simulink model "TV_FLC_V3_Codegen"  (R2026a)
settings: Solver=FixedStepDiscrete  StopTime=100  FixedStep=0.003  MaxStep=0.4  AbsTol=1e-3
model workspace (MAT data in the model file):
  Af = 1.20000004768
  C_alpha_F = 46504
  D = 11
  F = 0.0421790704131
  FIS_DYC_3 : fistree (value not decoded)
  Gain = 0.175131350756
  Gr = 5
  I = 6000
  Kp_TV_Beta : Simulink.Parameter (value not decoded)
  Kp_TV_Yaw : Simulink.Parameter (value not decoded)
  Ku = -0.000124337399029
  L = 1.57799994946
  Load_Ref = [0 400 500 600 700 800 900 1000 1100 1200 1300 1400 ... (18 elements, 18x1)]
  MotorT = [51.0306892395 51.0306892395 51.0306892395 51.0306892395 51.0306892395 51.0306892395 51.0306892395 51.0306892395 51.0306892395 51.0306892395 51.0306892395 51.0306892395 ... (47 elements, 1x47)]
  MotorW = [0 100 200 300 400 500 600 700 800 900 1000 1100 ... (47 elements, 1x47)]
  P = 800
  Slip_Ctrl_Kd : Simulink.Parameter (value not decoded)
  Slip_Ctrl_Ki : Simulink.Parameter (value not decoded)
  Slip_Ctrl_Kn : Simulink.Parameter (value not decoded)
  Slip_Ctrl_Kp : Simulink.Parameter (value not decoded)
  Slip_Ref = [0.151999995112 0.151999995112 0.151999995112 0.115999996662 0.101999998093 0.0960000008345 0.0920000001788 0.0900000035763 0.0900000035763 0.0900000035763 0.0939999967813 0.097999997437 ... (18 elements, 18x1)]
  Slip_Steer_th : Simulink.Parameter (value not decoded)
  Slip_TC_Enable : Simulink.Parameter (value not decoded)
  Tmax = 51.0306892395
  a = 0.823199987411
  a_cop = 0.707000017166
  cd = -2.15000009537
  g = 9.81000041962
  h_CG = 0.358300000429
  m = 320
  ro = 1.22599995136
  rwheel = 0.263000011444
  tr = 1.24800002575
  vx_th = 1
symbols that are objects in the model workspace (value not decoded): Kp_TV_Beta, Kp_TV_Yaw, Slip_Ctrl_Kd, Slip_Ctrl_Ki, Slip_Ctrl_Kn, Slip_Ctrl_Kp, Slip_Steer_th, Slip_TC_Enable
undefined symbols (not defined in the file or in its folder): dspblkCoreblockFVToolHelper, gcbh
libraries: simulink x5, sl_discontinuities x3, slpidlib x2, fuzblock x1
(part 2 of 2)

== system TV_FLC_V3_Codegen/Slip Control/Maximum Torque Allowed/Slip Correction Right ==
  Fz_rl : Inport  OutDataTypeStr=single
  kappa_rr : Inport  Port=2
  1-D Lookup Table : Lookup_n-D  NumberOfTableDimensions=1  BreakpointsForDimension1=Load_Ref  Table=Slip_Ref  ExtrapMethod=Clip  UseLastTableValue=on  InternalRulePriority=Speed  RndMeth=Simplest
  PID Controller : slpidlib/PID Controller  Controller=PID  Form=Parallel  TimeDomain=Discrete-time  UseExternalTs=off  SampleTime=0.003  IntegratorMethod=Forward Euler  FilterMethod=Forward Euler  ControllerParametersSource=internal  P=Slip_Ctrl_Kp  I=Slip_Ctrl_Ki  UseKiTs=off  D=Slip_Ctrl_Kd  UseExternalDerivativeSource=off  N=Slip_Ctrl_Kn  UseFilter=on  TunerSelectOption=Transfer Function Based (PID Tuner App)  InitialConditionSource=internal  InitialConditionForIntegrator=Tmax  InitialConditionForFilter=0  DifferentiatorICPrevScaledInput=Tmax  ExternalReset=none  TrackingMode=off  Kt=1  LimitOutput=on  SatLimitsSource=internal  UpperSaturationLimit=Tmax  LowerSaturationLimit=0  LinearizeAsGain=on  AntiWindupMode=clamping  Kb=1  LimitIntegrator=off  UpperIntegratorSaturationLimit=inf  LowerIntegratorSaturationLimit=-inf  POutMin=[]  POutMax=[]  IOutMin=[]  IOutMax=[]  DOutMin=[]  DOutMax=[]  NOutMin=[]  NOutMax=[]  SumOutMin=[]  SumOutMax=[]  SaturationOutMin=[]  SaturationOutMax=[]  PParamMin=[]  PParamMax=[]  IParamMin=[]  IParamMax=[]  DParamMin=[]  DParamMax=[]  NParamMin=[]  NParamMax=[]  KbParamMin=[]  KbParamMax=[]  KtParamMin=[]  KtParamMax=[]  KbOutMin=[]  KbOutMax=[]  KtOutMin=[]  KtOutMax=[]  IntegratorOutMin=[]  IntegratorOutMax=[]  FilterOutMin=[]  FilterOutMax=[]  SumI1OutMin=[]  SumI1OutMax=[]  SumI2OutMin=[]  SumI2OutMax=[]  SumI3OutMin=[]  SumI3OutMax=[]  SumI4OutMin=[]  SumI4OutMax=[]  SumDOutMin=[]  SumDOutMax=[]  DifferentiatorOutMin=[]  DifferentiatorOutMax=[]  FilterDiffOutCoefMin=[]  FilterDiffOutCoefMax=[]  ReciprocalOutMin=[]  ReciprocalOutMax=[]  SumDenOutMin=[]  SumDenOutMax=[]  SumNumOutMin=[]  SumNumOutMax=[]  DivideOutMin=[]  DivideOutMax=[]  UdiffTsProdOutMin=[]  UdiffTsProdOutMax=[]  NTsProdOutMin=[]  NTsProdOutMax=[]  UintegralTsProdOutMin=[]  UintegralTsProdOutMax=[]  UngainTsProdOutMin=[]  UngainTsProdOutMax=[]  ClampingZeroOutDataTypeStr=Inherit: Inherit via back propagation  ClampingZeroOutMin=[]  ClampingZeroOutMax=[]  FilterDenConstantOutDataTypeStr=Inherit: Inherit via back propagation  FilterDenConstantOutMin=[]  FilterDenConstantOutMax=[]  PCopyOutDataTypeStr=Inherit: Inherit via back propagation  PCopyOutMin=[]  PCopyOutMax=[]  NCopyOutDataTypeStr=Inherit: Inherit via back propagation  NCopyOutMin=[]  NCopyOutMax=[]  IntegratorContinuousStateAttributes=''  IntegratorStateMustResolveToSignalObject=off  IntegratorRTWStateStorageClass=Auto  FilterContinuousStateAttributes=''  FilterStateMustResolveToSignalObject=off  FilterRTWStateStorageClass=Auto  ParallelPVariant=InternalParameters  IdealPVariant=Disabled  IVariant=InternalParameters  DVariant=InternalParameters  IntegratorVariant=Discrete  SatVariant=Enabled  AWVariant=DiscClampingParallel  PCopyVariant=Disabled  TRVariant=Disabled  FdbkBlocksVariant=Forward  IdealPFdbkVariant=Disabled  SatFdbkVariant=Disabled  DerivativeFilterVariant=ForwardEulerFilter  NVariant=InternalParameters  NCopyVariant=Disabled  FilterICVariant=InternalICsFilter  IntegratorICVariant=InternalICs  ExternalResetVariant=Disabled  TRSumVariant=Passthrough  SumFdbkVariant=Disabled  SumVariant=Sum_PID  TsampFilterVariant=InternalTs  TsampNgainVariant=Passthrough  TsampIntegralVariant=Disabled_SignalSpec  ExternalSaturationOutDataTypeStr=Inherit: Same as second input  DerivativeSourceVariant=ErrorSignal  PreIntVariant=InternalPreInt
  Sum : Sum  Inputs=|+-
  Tmax_rr : Outport
  Out Bus Element : Outport  Port=2  PortName=Debug  Element=kappa_rr_ref
  wires:
  1-D Lookup Table/1 -> Out Bus Element/1, Sum/1  "kappa_ref"
  PID Controller/1 -> Tmax_rr/1  "Tmax_rl_Nm"
  kappa_rr/1 -> Sum/2  "kappa_rr"
  Sum/1 -> PID Controller/1  "e"
  Fz_rl/1 -> 1-D Lookup Table/1  "Fz_rr_N"

== system TV_FLC_V3_Codegen/Slip Control/Slip Calculation/Wheel Vx ==
  Vx : Inport
  nYaw : Inport  Port=2
  Add : Sum  Inputs=+-
  Add2 : Sum
  Divide : Product  Inputs=**
  Gain : Gain  Gain=1/2
  Rear Track : Constant  Value=tr  OutDataTypeStr=single
  vx_whl_rl : Outport
  vx_whl_rr : Outport  Port=2
  wires:
  Rear Track/1 -> Gain/1  "tr_m"
  nYaw/1 -> Divide/1  "nYaw_rad/s"
  Gain/1 -> Divide/2
  Vx/1 -> Add2/1, Add/1  "vx_m/s"
  Divide/1 -> Add2/2, Add/2
  Add/1 -> vx_whl_rl/1  "vx_whl_rl"
  Add2/1 -> vx_whl_rr/1  "vx_whl_rr"

== system TV_FLC_V3_Codegen/TV/Yaw Moment Required/Deadband Safety ==
  e_yaw_norm : Inport
  de_yaw_norm : Inport  Port=2
  Abs de_yaw : Abs
  Abs e_yaw : Abs
  Both small : Logic  AllPortsSameDT=off  OutDataTypeStr=boolean
  Switch de_yaw : Switch  Threshold=0.5  ZeroCross=off
  Switch e_yaw : Switch  Threshold=0.5  ZeroCross=off
  Zero de_yaw : Constant  Value=0  OutDataTypeStr=single  SampleTime=0.003
  Zero e_yaw : Constant  Value=0  OutDataTypeStr=single  SampleTime=0.003
  de_yaw below deadband : simulink/Logic and Bit Operations/Compare To Constant  relop=<  const=5e-2  OutDataTypeStr=boolean  ZeroCross=off
  e_yaw below deadband : simulink/Logic and Bit Operations/Compare To Constant  relop=<  const=1e-1  OutDataTypeStr=boolean  ZeroCross=off
  e_yaw_safe : Outport
  de_yaw_safe : Outport  Port=2
  wires:
  e_yaw_norm/1 -> Switch e_yaw/3, Abs e_yaw/1
  de_yaw_norm/1 -> Switch de_yaw/3, Abs de_yaw/1
  Switch de_yaw/1 -> de_yaw_safe/1
  Abs de_yaw/1 -> de_yaw below deadband/1
  Switch e_yaw/1 -> e_yaw_safe/1
  Abs e_yaw/1 -> e_yaw below deadband/1
  e_yaw below deadband/1 -> Both small/1
  de_yaw below deadband/1 -> Both small/2
  Zero de_yaw/1 -> Switch de_yaw/1
  Zero e_yaw/1 -> Switch e_yaw/1
  Both small/1 -> Switch e_yaw/2, Switch de_yaw/2

== matlab function TV_FLC_V3_Codegen/TV/Yaw Moment Required/MATLAB Function ==
  data: delta_SW input; s_turn output; delta_th parameter
function s_turn = fcn(delta_SW, delta_th)
delta_th = deg2rad(delta_th);
if delta_SW >= delta_th
    s_turn = single(+1);
elseif delta_SW <= -delta_th
    s_turn = single(-1);
elseif abs(delta_SW) < delta_th
    s_turn = single(0);
else
    s_turn = single(0);
end

end

== matlab function TV_FLC_V3_Codegen/Slip Activation/MATLAB Function ==
  data: aSteerWheel input; ay input; steer_th input; nYaw input; slip_active output single; slip_active_previous input
function slip_active = fcn(aSteerWheel, ay, steer_th, nYaw,slip_active_previous)
ay_on = 0.2*9.81;
ay_off = 0.1 * 9.81;
r_on = 0.15;
r_off = 0.08;
steer_th_on = deg2rad(steer_th);
steer_th_off = deg2rad(steer_th)/2;
on_cond = abs(aSteerWheel) > steer_th_on || ...
    abs(ay)          > ay_on    || ...
    abs(nYaw)        > r_on;

off_cond = abs(aSteerWheel) < steer_th_off && ...
    abs(ay)          < ay_off    && ...
    abs(nYaw)        < r_off;

if on_cond
    slip_active = single(1);
elseif off_cond
    slip_active = single(0);
else
    slip_active = slip_active_previous;
end

end
